simulink model "Three_Phase_Four_Leg_Inverter"  (R2023b)
settings: Solver=FixedStepAuto  StartTime=0.0  StopTime=0.5  RelTol=1e-3
libraries: spsSeriesRLCBranchLib x11, spsVoltageMeasurementLib x7, spsUniversalBridgeLib x4, spsDCVoltageSourceLib x3, spsCurrentMeasurementLib x3, spsRMSLib x2, simulink x1, spsMeanLib x1, spsTHDLib x1, spspowerguiLib x1
settings Model: SimulationMode=accelerator  Creator=abc6820292  LastModifiedBy=Qu
settings SolverCC: ZeroCrossAlgorithm=Adaptive
settings DataIOCC: ReturnWorkspaceOutputs=off  Refine=10
settings DebuggingCC: IgnoredZcDiagnostic=none  UnconnectedInputMsg=warning  UnconnectedOutputMsg=warning  UnconnectedLineMsg=warning
settings ModelReferenceCC: EnableRefExpFcnMdlSchedulingChecks=on
settings RTWCC: DLArmComputeVersion=19.05

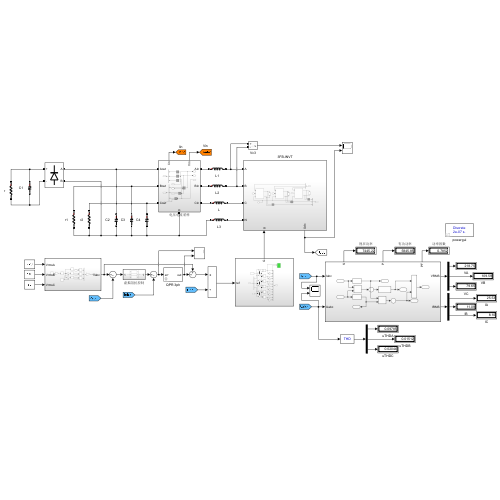
[thumbnail: Simulink's stored preview of the top-level diagram]
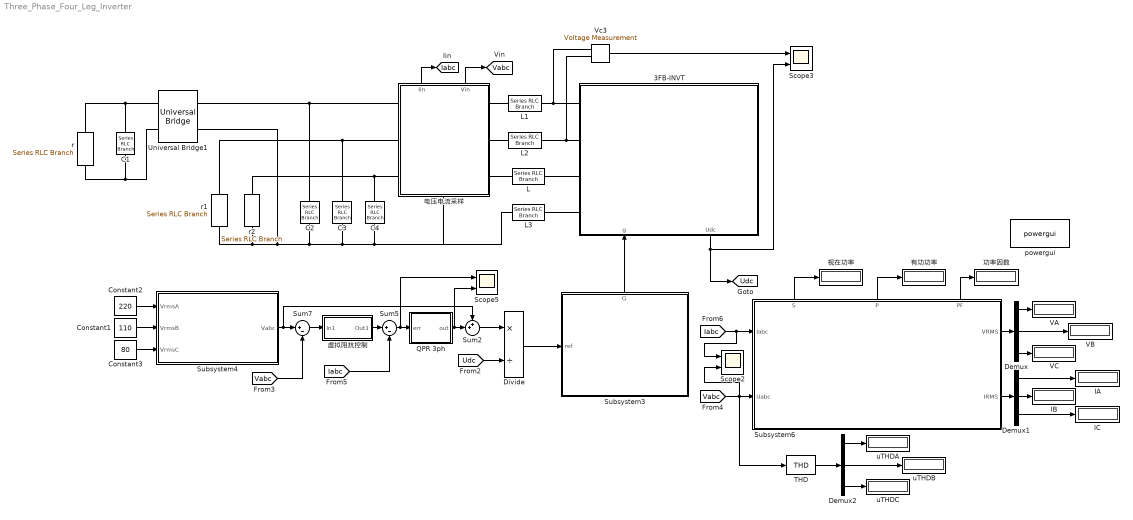
== system Three_Phase_Four_Leg_Inverter ==
  3FB-INVT : Subsystem
      settings: PortSchema="{\"entries\":[{\"content\":{\"sides\":[{\"content\":{\"connectorIds\":[\"LConn1\",\"LConn2\",\"LConn3\",\"LConn4\"]},\"type\":\"ConnectorPlacement.EquallySpacedRectSide\",\"uuid\":\"b14efc91-6835-4ed7-8c1d-e2670cf7c179\"},{\"content\":{\"side\":\"RIGHT\"},\"type\":\"ConnectorPlacement.EquallySpacedRectSide\",\"uuid\":\"133f26b8-b252-4d3c-80df-0b09760e0c14\"},{\"content\":{\"side\":\"TOP\"},\"type\":\"ConnectorPlacement.EquallySpacedRectSide\",\"uuid\":\"c058e102-7791-48c2-b9e4-e80cedcfd34e\"},{\"content\":{\"connectorIds\":[\"In1\",\"Out1\"],\"side\":\"BOTTOM\"},\"type\":\"ConnectorPlacement.EquallySpacedRectSide\",\"uuid\":\"7bcd8845-3331-4b31-8039-611891643c20\"}]},\"type\":\"ConnectorPlacement.EquallySpacedConnector\",\"uuid\":\"173e4324-58a1-473c-9df3-d0606e4a673f\"}],\"packageUris\":[\"http://schema.mathworks.com/mf0/Connector/R2020b\"],\"version\":\"1.0\"}"
  C1 : spsSeriesRLCBranchLib/Series RLC Branch  LConnTagsString=__new0  RConnTagsString=__new0  BranchType=C  Resistance=0  Inductance=0  SetiL0=off  InitialCurrent=0  Capacitance=5e-3  Setx0=on  InitialVoltage=310  Measurements=None
  C2 : spsSeriesRLCBranchLib/Series RLC Branch  LConnTagsString=__new0  RConnTagsString=__new0  BranchType=C  Resistance=0  Inductance=0  SetiL0=off  InitialCurrent=0  Capacitance=5e-6  Setx0=off  InitialVoltage=310  Measurements=None
  C3 : spsSeriesRLCBranchLib/Series RLC Branch  LConnTagsString=__new0  RConnTagsString=__new0  BranchType=C  Resistance=0  Inductance=0  SetiL0=off  InitialCurrent=0  Capacitance=5e-6  Setx0=off  InitialVoltage=310  Measurements=None
  C4 : spsSeriesRLCBranchLib/Series RLC Branch  LConnTagsString=__new0  RConnTagsString=__new0  BranchType=C  Resistance=0  Inductance=0  SetiL0=off  InitialCurrent=0  Capacitance=5e-6  Setx0=off  InitialVoltage=310  Measurements=None
  Constant1 : Constant  Value=110
  Constant2 : Constant  Value=220
  Constant3 : Constant  Value=80
  Demux : Demux  Outputs=3
  Demux1 : Demux  Outputs=3
  Demux2 : Demux  Outputs=3
  Divide : Product  Inputs=*/
  IA : Display
      settings: Format=bank
  IB : Display
      settings: Format=bank
  IC : Display
      settings: Format=bank
  L : spsSeriesRLCBranchLib/Series RLC Branch  LConnTagsString=__new0  RConnTagsString=__new0  BranchType=L  Resistance=1  Inductance=2e-4  SetiL0=off  InitialCurrent=0  Capacitance=inf  Setx0=off  InitialVoltage=0  Measurements=None
  L1 : spsSeriesRLCBranchLib/Series RLC Branch  LConnTagsString=__new0  RConnTagsString=__new0  BranchType=L  Resistance=1  Inductance=2e-4  SetiL0=off  InitialCurrent=0  Capacitance=inf  Setx0=off  InitialVoltage=0  Measurements=None
  L2 : spsSeriesRLCBranchLib/Series RLC Branch  LConnTagsString=__new0  RConnTagsString=__new0  BranchType=L  Resistance=1  Inductance=2e-4  SetiL0=off  InitialCurrent=0  Capacitance=inf  Setx0=off  InitialVoltage=0  Measurements=None
  L3 : spsSeriesRLCBranchLib/Series RLC Branch  LConnTagsString=__new0  RConnTagsString=__new0  BranchType=L  Resistance=0.01  Inductance=2e-4  SetiL0=off  InitialCurrent=0  Capacitance=inf  Setx0=off  InitialVoltage=0  Measurements=None
  QPR 3ph : Subsystem  mask{Kp=8, Kr=100, Wc=5, Ts=1/30000, Upper=600, Lower=-600}
      mask DialogControl ParameterGroupVar Prompt: 参数
  Scope2 : Scope  NumInputPorts=2
  Scope3 : Scope  NumInputPorts=2
  Scope5 : Scope  NumInputPorts=2
  Subsystem3 : Subsystem
      settings: PortSchema="{\"entries\":[{\"content\":{\"sides\":[{\"content\":{\"connectorIds\":[\"In1\"]},\"type\":\"ConnectorPlacement.EquallySpacedRectSide\",\"uuid\":\"86d8a801-af54-4615-919a-9a70996995f5\"},{\"content\":{\"side\":\"RIGHT\"},\"type\":\"ConnectorPlacement.EquallySpacedRectSide\",\"uuid\":\"9c099dd5-197a-4a29-8cd5-6822de601230\"},{\"content\":{\"connectorIds\":[\"Out1\"],\"side\":\"TOP\"},\"type\":\"ConnectorPlacement.EquallySpacedRectSide\",\"uuid\":\"5852d946-2383-4602-be71-32d16fa24bc3\"}]},\"type\":\"ConnectorPlacement.EquallySpacedConnector\",\"uuid\":\"a21c857f-e780-49b2-9a65-1676cf4540b1\"}],\"packageUris\":[\"http://schema.mathworks.com/mf0/Connector/R2020b\"],\"version\":\"1.0\"}"
  Subsystem4 : Subsystem
  Subsystem6 : Subsystem
      settings: PortSchema="{\"entries\":[{\"content\":{\"sides\":[{\"content\":{\"connectorIds\":[\"In1\",\"In2\"]},\"type\":\"ConnectorPlacement.EquallySpacedRectSide\",\"uuid\":\"8f3b7bf1-7c44-4492-a357-aa6e3e6d66a4\"},{\"content\":{\"connectorIds\":[\"Out1\",\"Out2\"],\"side\":\"RIGHT\"},\"type\":\"ConnectorPlacement.EquallySpacedRectSide\",\"uuid\":\"7ae784cf-6bcf-4684-9c07-1770fc60c8a0\"},{\"content\":{\"connectorIds\":[\"Out3\",\"Out4\",\"Out5\"],\"side\":\"TOP\"},\"type\":\"ConnectorPlacement.EquallySpacedRectSide\",\"uuid\":\"0e016931-6232-4ad6-afe9-572a0571336f\"},{\"content\":{\"side\":\"BOTTOM\"},\"type\":\"ConnectorPlacement.EquallySpacedRectSide\",\"uuid\":\"ef67c6ee-ba81-4705-af34-81581e7e9907\"}]},\"type\":\"ConnectorPlacement.EquallySpacedConnector\",\"uuid\":\"922af512-c0ff-443f-816c-194775a78dc8\"}],\"packageUris\":[\"http://schema.mathworks.com/mf0/Connector/R2020b\"],\"version\":\"1.0\"}"
  Sum2 : Sum  Inputs=++|
  Sum5 : Sum  Inputs=|+-
  Sum7 : Sum  Inputs=|+-
  THD : spsTHDLib/THD  Freq=50  Ts=0
  Universal Bridge1 : spsUniversalBridgeLib/Universal Bridge  Arms=2  SnubberResistance=1e6  SnubberCapacitance=inf  Device=Diodes  Ron=1e-3  Lon=0  ForwardVoltages="[  1  1  ]"  ForwardVoltage=1  GTOparameters=[ 10e-6 , 20e-6 ]  IGBTparameters=[ 1e-6 , 2e-6 ]  Measurements=None  Measurements_2=None  converterType=Rectifier
  VA : Display
      settings: Format=bank
  VB : Display
      settings: Format=bank
  VC : Display
      settings: Format=bank
  Vc3 : spsVoltageMeasurementLib/Voltage Measurement  PhasorSimulation=off  OutputType=Complex  PSBequivalent=0
  powergui : spspowerguiLib/powergui  Priority=1  SimulationMode=Discrete  SampleTime=2e-7  frequency=60  Iterations=50  frequencyindice=0  Pbase=100e6  ErrMax=1e-4  UnitsV=kV  UnitsW=MW  buscounter=0  FunctionMessages=off  echomessages=off  EnableUseOfTLC=off  CurrentSourceSwitches=off  DisableSnubberDevices=off  DisableRonSwitches=off  DisableVfSwitches=off  DisplayEquations=off  AutomaticDiscreteSolvers=off  SolverType=Tustin/Backward Euler (TBE)  Interpol=off  ExternalGateDelay=off  methode=off  Ts=100  x0status=blocks  SPID=on  SwTol=0  HookPort=off  NonlinearTolerance=1e-4  nMaxIteration=100  ContinueOnMaxIteration=off  RestoreLinks=warning  ResistiveCurrentMeasurement=off  Frange=[0:2:500]  Ylog=off  Xlog=on  ShowGrid=off  save=off  variable=ZData  structure=0  ZoomFFT=off  StartTime=0.0  cycles=1  DisplayStyle=1  fundamental=60  FreqAxis=off  MaxFrequency=1000  frequencyindicesteady=1  RmsSteady=1  display=off
  r : spsSeriesRLCBranchLib/Series RLC Branch  LConnTagsString=__new0  RConnTagsString=__new0  BranchType=R  Resistance=30  Inductance=12e-4  SetiL0=off  InitialCurrent=0  Capacitance=inf  Setx0=off  InitialVoltage=0  Measurements=None
  r1 : spsSeriesRLCBranchLib/Series RLC Branch  LConnTagsString=__new0  RConnTagsString=__new0  BranchType=R  Resistance=10  Inductance=12e-4  SetiL0=off  InitialCurrent=0  Capacitance=inf  Setx0=off  InitialVoltage=0  Measurements=None
  r2 : spsSeriesRLCBranchLib/Series RLC Branch  LConnTagsString=__new0  RConnTagsString=__new0  BranchType=R  Resistance=10  Inductance=12e-4  SetiL0=off  InitialCurrent=0  Capacitance=inf  Setx0=off  InitialVoltage=0  Measurements=None
  uTHDA : Display
  uTHDB : Display
  uTHDC : Display
  功率因数 : Display
  有功功率 : Display
      settings: Format=bank
  电压电流采样 : Subsystem
      settings: PortSchema="{\"entries\":[{\"content\":{\"sides\":[{\"content\":{\"connectorIds\":[\"LConn1\",\"LConn2\",\"LConn3\"]},\"type\":\"ConnectorPlacement.EquallySpacedRectSide\",\"uuid\":\"d60dd16a-7a74-435a-96f5-79c0993f3801\"},{\"content\":{\"connectorIds\":[\"RConn1\",\"RConn2\",\"RConn3\"],\"side\":\"RIGHT\"},\"type\":\"ConnectorPlacement.EquallySpacedRectSide\",\"uuid\":\"38a0d536-50a5-43bd-9d58-6b0db9c378a0\"},{\"content\":{\"connectorIds\":[\"Out1\",\"Out2\"],\"side\":\"TOP\"},\"type\":\"ConnectorPlacement.EquallySpacedRectSide\",\"uuid\":\"65be575f-dbb8-4f94-beb1-b426df65c1d5\"},{\"content\":{\"connectorIds\":[\"RConn4\"],\"side\":\"BOTTOM\"},\"type\":\"ConnectorPlacement.EquallySpacedRectSide\",\"uuid\":\"a28dffe8-15db-4523-b673-2414d0fbe1e1\"}]},\"type\":\"ConnectorPlacement.EquallySpacedConnector\",\"uuid\":\"1fc3ca7a-50b1-4fd5-a5d3-d39cc1e6f07d\"}],\"packageUris\":[\"http://schema.mathworks.com/mf0/Connector/R2020b\"],\"version\":\"1.0\"}"
  虚拟阻抗控制 : Subsystem
  视在功率 : Display
      settings: Format=bank
  tag scope: Iabc=global, Udc=global, Vabc=global
  wires:
  Vc3/1 -> Scope3/1
  3FB-INVT/1(Udc) -> [Udc], Scope3/2
  Subsystem3/1(G) -> 3FB-INVT/1(g)
  Demux/3 -> VC/1
  [Udc] -> Divide/2
  Sum2/1 -> Divide/1
  Demux2/1 -> uTHDA/1
  Subsystem6/3(S) -> 视在功率/1
  Demux/1 -> VA/1
  [Vabc] -> THD/1, Scope2/2, Subsystem6/2(Uabc)
  Subsystem6/1(VRMS) -> Demux/1
  QPR 3ph/1(out) -> Scope5/2, Sum2/2
  Demux2/3 -> uTHDC/1
  Demux1/1 -> IA/1
  Divide/1 -> Subsystem3/1(ref)
  Demux/2 -> VB/1
  Demux1/3 -> IC/1
  虚拟阻抗控制/1(Out1) -> Sum5/1
  THD/1 -> Demux2/1
  Subsystem6/5(PF) -> 功率因数/1
  Subsystem6/4(P) -> 有功功率/1
  Demux2/2 -> uTHDB/1
  Demux1/2 -> IB/1
  Subsystem4/1(Vabc) -> Sum2/1, Sum7/1
  Subsystem6/2(IRMS) -> Demux1/1
  [Iabc] -> Scope2/1, Subsystem6/1(Iabc)
  Sum5/1 -> Scope5/1, QPR 3ph/1(err)
  Constant2/1 -> Subsystem4/1(VrmsA)
  Sum7/1 -> 虚拟阻抗控制/1(In1)
  [Vabc] -> Sum7/2
  [Iabc] -> Sum5/2
  电压电流采样/1(Vin) -> [Vabc]
  电压电流采样/2(Iin) -> [Iabc]
  Constant1/1 -> Subsystem4/2(VrmsB)
  Constant3/1 -> Subsystem4/3(VrmsC)
  connections:
  C3/LConn1 -- 电压电流采样/RConn2 -- r1/LConn1
  r2/RConn1 -- r1/RConn1 -- Universal Bridge1/LConn2 -- C4/RConn1 -- 电压电流采样/RConn4 -- L3/LConn1 -- C3/RConn1 -- C2/RConn1
  L1/RConn1 -- Vc3/LConn1 -- 3FB-INVT/LConn1
  C2/LConn1 -- 电压电流采样/RConn1 -- Universal Bridge1/LConn1
  L2/RConn1 -- Vc3/LConn2 -- 3FB-INVT/LConn2
  C4/LConn1 -- 电压电流采样/RConn3 -- r2/LConn1
  电压电流采样/LConn2 -- L2/LConn1
  L/RConn1 -- 3FB-INVT/LConn3
  电压电流采样/LConn1 -- L1/LConn1
  电压电流采样/LConn3 -- L/LConn1
  L3/RConn1 -- 3FB-INVT/LConn4
  Universal Bridge1/RConn1 -- C1/LConn1 -- r/LConn1
  Universal Bridge1/RConn2 -- C1/RConn1 -- r/RConn1

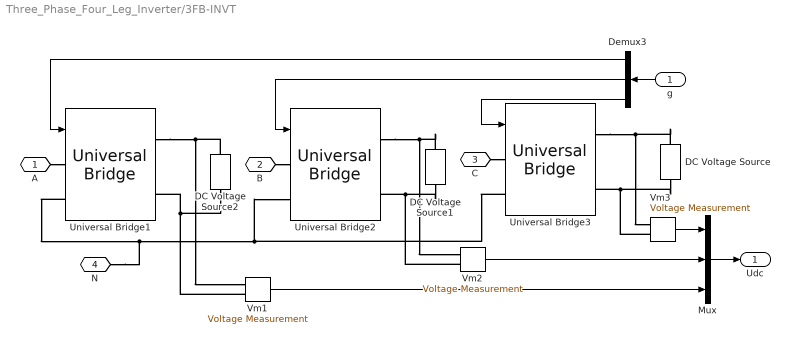
== system Three_Phase_Four_Leg_Inverter/3FB-INVT ==
  g : Inport
  DC Voltage Source : spsDCVoltageSourceLib/DC Voltage Source  Amplitude=375  Measurements=None
  DC Voltage Source1 : spsDCVoltageSourceLib/DC Voltage Source  Amplitude=375  Measurements=None
  DC Voltage Source2 : spsDCVoltageSourceLib/DC Voltage Source  Amplitude=375  Measurements=None
  Demux3 : Demux  Outputs=3
  Mux : Mux  Inputs=3
  Universal Bridge1 : spsUniversalBridgeLib/Universal Bridge  Arms=2  SnubberResistance=1e6  SnubberCapacitance=inf  Device=IGBT / Diodes  Ron=1e-3  Lon=0  ForwardVoltages="[  1  1  ]"  ForwardVoltage=0  GTOparameters=[ 10e-6 , 20e-6 ]  IGBTparameters=[ 1e-6 , 2e-6 ]  Measurements=None  Measurements_2=None  converterType=Rectifier
  Universal Bridge2 : spsUniversalBridgeLib/Universal Bridge  Arms=2  SnubberResistance=1e6  SnubberCapacitance=inf  Device=IGBT / Diodes  Ron=1e-3  Lon=0  ForwardVoltages="[  1  1  ]"  ForwardVoltage=0  GTOparameters=[ 10e-6 , 20e-6 ]  IGBTparameters=[ 1e-6 , 2e-6 ]  Measurements=None  Measurements_2=None  converterType=Rectifier
  Universal Bridge3 : spsUniversalBridgeLib/Universal Bridge  Arms=2  SnubberResistance=1e6  SnubberCapacitance=inf  Device=IGBT / Diodes  Ron=1e-3  Lon=0  ForwardVoltages="[  1  1  ]"  ForwardVoltage=0  GTOparameters=[ 10e-6 , 20e-6 ]  IGBTparameters=[ 1e-6 , 2e-6 ]  Measurements=None  Measurements_2=None  converterType=Rectifier
  Vm1 : spsVoltageMeasurementLib/Voltage Measurement  PhasorSimulation=off  OutputType=Complex  PSBequivalent=0
  Vm2 : spsVoltageMeasurementLib/Voltage Measurement  PhasorSimulation=off  OutputType=Complex  PSBequivalent=0
  Vm3 : spsVoltageMeasurementLib/Voltage Measurement  PhasorSimulation=off  OutputType=Complex  PSBequivalent=0
  A : PMIOPort  Side=Left
  B : PMIOPort  Port=2  Side=Left
  C : PMIOPort  Port=3  Side=Left
  N : PMIOPort  Port=4  Side=Left
  Udc : Outport
  wires:
  g/1 -> Demux3/1
  Vm3/1 -> Mux/1
  Vm2/1 -> Mux/2
  Vm1/1 -> Mux/3
  Demux3/3 -> Universal Bridge3/1
  Demux3/2 -> Universal Bridge2/1
  Demux3/1 -> Universal Bridge1/1
  Mux/1 -> Udc/1
  connections:
  Universal Bridge1/RConn1 -- DC Voltage Source2/RConn1 -- Vm1/LConn1
  Vm1/LConn2 -- Universal Bridge1/RConn2 -- DC Voltage Source2/LConn1
  A/RConn1 -- Universal Bridge1/LConn1
  Universal Bridge2/RConn1 -- DC Voltage Source1/RConn1 -- Vm2/LConn1
  Vm2/LConn2 -- DC Voltage Source1/LConn1 -- Universal Bridge2/RConn2
  Universal Bridge3/RConn1 -- DC Voltage Source/RConn1 -- Vm3/LConn1
  Vm3/LConn2 -- Universal Bridge3/RConn2 -- DC Voltage Source/LConn1
  B/RConn1 -- Universal Bridge2/LConn1
  C/RConn1 -- Universal Bridge3/LConn1
  Universal Bridge1/LConn2 -- N/RConn1 -- Universal Bridge3/LConn2 -- Universal Bridge2/LConn2

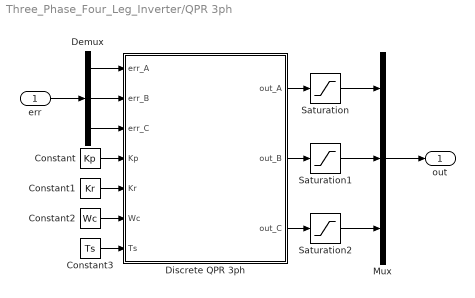
== system Three_Phase_Four_Leg_Inverter/QPR 3ph ==
  err : Inport
  Constant : Constant  Value=Kp
  Constant1 : Constant  Value=Kr
  Constant2 : Constant  Value=Wc
  Constant3 : Constant  Value=Ts
  Demux : Demux  Outputs=3
  Discrete QPR 3ph : MATLAB Function  TreatAsAtomicUnit=on
  Mux : Mux  Inputs=3
  Saturation : Saturate  UpperLimit=Upper  LowerLimit=Lower
  Saturation1 : Saturate  UpperLimit=Upper  LowerLimit=Lower
  Saturation2 : Saturate  UpperLimit=Upper  LowerLimit=Lower
  out : Outport
  wires:
  Discrete QPR 3ph/1(out_A) -> Saturation/1
  Constant1/1 -> Discrete QPR 3ph/5(Kr)
  Constant3/1 -> Discrete QPR 3ph/7(Ts)
  Constant/1 -> Discrete QPR 3ph/4(Kp)
  Constant2/1 -> Discrete QPR 3ph/6(Wc)
  Discrete QPR 3ph/2(out_B) -> Saturation1/1
  Discrete QPR 3ph/3(out_C) -> Saturation2/1
  Demux/2 -> Discrete QPR 3ph/2(err_B)
  Demux/3 -> Discrete QPR 3ph/3(err_C)
  Demux/1 -> Discrete QPR 3ph/1(err_A)
  err/1 -> Demux/1
  Saturation2/1 -> Mux/3
  Saturation1/1 -> Mux/2
  Saturation/1 -> Mux/1
  Mux/1 -> out/1

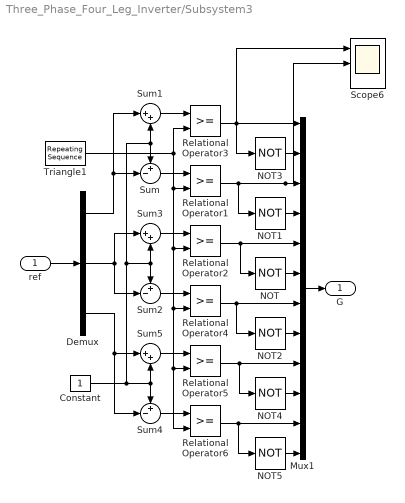
== system Three_Phase_Four_Leg_Inverter/Subsystem3 ==
  ref : Inport
  Constant : Constant
  Demux : Demux  Outputs=3
  Mux1 : Mux  Inputs=12
  NOT{,1..5} (6 alike) : Logic  Operator=NOT  IconShape=distinctive  AllPortsSameDT=off  OutDataTypeStr=boolean
  Relational Operator{1..6} (6 alike) : RelationalOperator  OutDataTypeStr=boolean  InputSameDT=off
  Scope6 : Scope  NumInputPorts=3
  Sum : Sum  Inputs=+-|
  Sum1 : Sum  Inputs=|++
  Sum2 : Sum  Inputs=+-|
  Sum3 : Sum  Inputs=|++
  Sum4 : Sum  Inputs=+-|
  Sum5 : Sum  Inputs=|++
  Triangle1 : simulink/Sources/Repeating Sequence  rep_seq_t=[0 1/30000/2 1/30000]  rep_seq_y=[0 2 0]
  G : Outport
  wires:
  Relational Operator2/1 -> Mux1/5, NOT/1
  Relational Operator3/1 -> NOT3/1, Scope6/1, Mux1/1
  Mux1/1 -> G/1
  Relational Operator5/1 -> Mux1/9, NOT4/1
  Relational Operator6/1 -> Mux1/11, NOT5/1
  NOT3/1 -> Mux1/2
  NOT/1 -> Mux1/6
  NOT4/1 -> Mux1/10
  Triangle1/1 -> Relational Operator6/2, Relational Operator5/2, Relational Operator4/2, Relational Operator2/2, Relational Operator1/2, Relational Operator3/2
  Sum/1 -> Relational Operator1/1
  Demux/1 -> Sum1/1, Sum/2
  Sum1/1 -> Relational Operator3/1
  Constant/1 -> Sum/1, Sum1/2, Sum3/2, Sum2/1, Sum5/2, Sum4/1
  Demux/2 -> Sum2/2, Sum3/1
  Sum3/1 -> Relational Operator2/1
  Sum2/1 -> Relational Operator4/1
  Sum5/1 -> Relational Operator5/1
  Sum4/1 -> Relational Operator6/1
  Demux/3 -> Sum4/2, Sum5/1
  NOT5/1 -> Mux1/12
  NOT2/1 -> Mux1/8
  Relational Operator4/1 -> NOT2/1, Mux1/7
  NOT1/1 -> Mux1/4
  Relational Operator1/1 -> Scope6/2, Mux1/3, NOT1/1
  ref/1 -> Demux/1

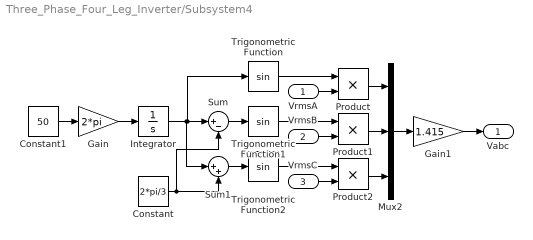
== system Three_Phase_Four_Leg_Inverter/Subsystem4 ==
  VrmsA : Inport
  VrmsB : Inport  Port=2
  VrmsC : Inport  Port=3
  Constant : Constant  Value=2*pi/3
  Constant1 : Constant  Value=50
  Gain : Gain  Gain=2*pi
  Gain1 : Gain  Gain=1.415
  Integrator : Integrator  WrapState=on  WrappedStateUpperValue=2*pi  WrappedStateLowerValue=0
  Mux2 : Mux  Inputs=3
  Product : Product
  Product1 : Product
  Product2 : Product
  Sum : Sum  Inputs=|+-
  Sum1 : Sum  Inputs=|++
  Trigonometric Function : Trigonometry
  Trigonometric Function1 : Trigonometry
  Trigonometric Function2 : Trigonometry
  Vabc : Outport
  wires:
  Gain/1 -> Integrator/1
  Integrator/1 -> Sum1/1, Trigonometric Function/1, Sum/1
  Constant/1 -> Sum1/2, Sum/2
  Sum/1 -> Trigonometric Function1/1
  Sum1/1 -> Trigonometric Function2/1
  Constant1/1 -> Gain/1
  Trigonometric Function/1 -> Product/1
  Product/1 -> Mux2/1
  Trigonometric Function1/1 -> Product1/1
  Product1/1 -> Mux2/2
  Trigonometric Function2/1 -> Product2/1
  Product2/1 -> Mux2/3
  Mux2/1 -> Gain1/1
  Gain1/1 -> Vabc/1
  VrmsA/1 -> Product/2
  VrmsC/1 -> Product2/2
  VrmsB/1 -> Product1/2

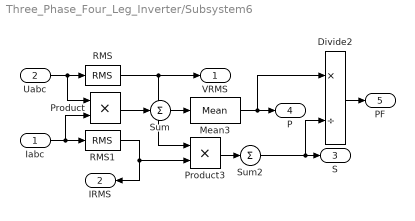
== system Three_Phase_Four_Leg_Inverter/Subsystem6 ==
  Iabc : Inport
  Uabc : Inport  Port=2
  Divide2 : Product  Inputs=*/
  Mean3 : spsMeanLib/Mean  Freq=50  Vinit=0  Ts=0
  Product : Product
  Product3 : Product
  RMS : spsRMSLib/RMS  TrueRMS=on  Freq=50  RMSInit=0  Ts=0
  RMS1 : spsRMSLib/RMS  TrueRMS=on  Freq=50  RMSInit=0  Ts=0
  Sum : Sum  Inputs=+
  Sum2 : Sum  Inputs=+
  VRMS : Outport
  IRMS : Outport  Port=2
  S : Outport  Port=3
  P : Outport  Port=4
  PF : Outport  Port=5
  wires:
  Iabc/1 -> Product/2, RMS1/1
  RMS/1 -> VRMS/1, Product3/1
  RMS1/1 -> Product3/2, IRMS/1
  Divide2/1 -> PF/1
  Mean3/1 -> Divide2/1, P/1
  Sum/1 -> Mean3/1
  Uabc/1 -> RMS/1, Product/1
  Product/1 -> Sum/1
  Product3/1 -> Sum2/1
  Sum2/1 -> Divide2/2, S/1

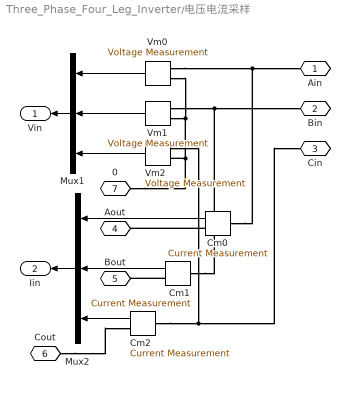
== system Three_Phase_Four_Leg_Inverter/电压电流采样 ==
  Cm0 : spsCurrentMeasurementLib/Current Measurement  PhasorSimulation=off  OutputType=Complex  PSBequivalent=0
  Cm1 : spsCurrentMeasurementLib/Current Measurement  PhasorSimulation=off  OutputType=Complex  PSBequivalent=0
  Cm2 : spsCurrentMeasurementLib/Current Measurement  PhasorSimulation=off  OutputType=Complex  PSBequivalent=0
  Mux1 : Mux  Inputs=3
  Mux2 : Mux  Inputs=3
  Vm0 : spsVoltageMeasurementLib/Voltage Measurement  PhasorSimulation=off  OutputType=Complex  PSBequivalent=0
  Vm1 : spsVoltageMeasurementLib/Voltage Measurement  PhasorSimulation=off  OutputType=Complex  PSBequivalent=0
  Vm2 : spsVoltageMeasurementLib/Voltage Measurement  PhasorSimulation=off  OutputType=Complex  PSBequivalent=0
  Ain : PMIOPort  Side=Left
  Bin : PMIOPort  Port=2  Side=Left
  Cin : PMIOPort  Port=3  Side=Left
  Aout : PMIOPort  Port=4  Side=Right
  Bout : PMIOPort  Port=5  Side=Right
  Cout : PMIOPort  Port=6  Side=Right
  0 : PMIOPort  Port=7  Side=Right
  Vin : Outport
  Iin : Outport  Port=2
  wires:
  Cm2/1 -> Mux2/3
  Vm1/1 -> Mux1/2
  Cm1/1 -> Mux2/2
  Vm2/1 -> Mux1/3
  Vm0/1 -> Mux1/1
  Mux1/1 -> Vin/1
  Cm0/1 -> Mux2/1
  Mux2/1 -> Iin/1
  connections:
  Vm1/LConn1 -- Cm1/LConn1 -- Bin/RConn1
  Cm0/RConn1 -- Aout/RConn1
  Vm0/LConn1 -- Cm0/LConn1 -- Ain/RConn1
  Cm2/LConn1 -- Vm2/LConn1 -- Cin/RConn1
  Cm1/RConn1 -- Bout/RConn1
  Cout/RConn1 -- Cm2/RConn1
  0/RConn1 -- Vm0/LConn2 -- Vm1/LConn2 -- Vm2/LConn2

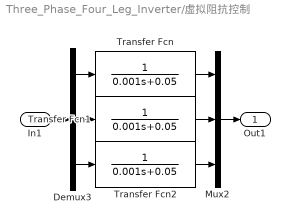
== system Three_Phase_Four_Leg_Inverter/虚拟阻抗控制 ==
  In1 : Inport
  Demux3 : Demux  Outputs=3
  Mux2 : Mux  Inputs=3
  Transfer Fcn : TransferFcn  Denominator=[0.001 0.05]
  Transfer Fcn1 : TransferFcn  Denominator=[0.001 0.05]
  Transfer Fcn2 : TransferFcn  Denominator=[0.001 0.05]
  Out1 : Outport
  wires:
  Demux3/2 -> Transfer Fcn1/1
  Transfer Fcn/1 -> Mux2/1
  Mux2/1 -> Out1/1
  Transfer Fcn1/1 -> Mux2/2
  Transfer Fcn2/1 -> Mux2/3
  Demux3/3 -> Transfer Fcn2/1
  Demux3/1 -> Transfer Fcn/1
  In1/1 -> Demux3/1

== matlab function Three_Phase_Four_Leg_Inverter/QPR 3ph/Discrete QPR 3ph ==
  settings: updateMethod=DISCRETE  sampleTime=Ts
  data: err_A input; err_B input; err_C input; out_A output; Kp input; Kr input; Wc input; Ts input; out_B output; out_C output
function [out_A, out_B, out_C] = fcn(err_A, err_B, err_C, Kp, Kr, Wc, Ts)

W0 = 50*2*pi;

%%定义三相静态变量
persistent err_A1;
persistent err_A2;
persistent out_A1;
persistent out_A2;

persistent err_B1;
persistent err_B2;
persistent out_B1;
persistent out_B2;

persistent err_C1;
persistent err_C2;
persistent out_C1;
persistent out_C2;

%%对三相静态变量初始化
if isempty(err_A1)
    err_A1 = 0;
end
if isempty(err_A2)
    err_A2 = 0;
end
if isempty(out_A1)
    out_A1 = 0;
end
if isempty(out_A2)
    out_A2 = 0;
end

if isempty(err_B1)
    err_B1 = 0;
end
if isempty(err_B2)
    err_B2 = 0;
end
if isempty(out_B1)
    out_B1 = 0;
end
if isempty(out_B2)
    out_B2 = 0;
end

if isempty(err_C1)
    err_C1 = 0;
end
if isempty(err_C2)
    err_C2 = 0;
end
if isempty(out_C1)
    out_C1 = 0;
end
if isempty(out_C2)
    out_C2 = 0;
end

%%Discrete
t1 = Wc * Ts;
t2 = W0^2 * Ts^2;
t3 = t2 + 4*t1 + 4;

b0 = (Kp*t2 + 4*(Kp+Kr)*t1 + 4*Kp) / t3;
b1 = (2*Kp*t2 - 8*Kp) / t3;
b2 = (Kp*t2 + 4*Kp - 4*(Kp+Kr)*t1) / t3;
a1 = (2*t2 - 8) / t3;
a2 = (t2 - 4*t1 + 4) / t3;

%%计算三相输出量
out_A = b0*err_A + b1*err_A1 + b2*err_A2 - a1*out_A1 - a2*out_A2;
out_A2 = out_A1;
out_A1 = out_A;
err_A2 = err_A1;
err_A1 = err_A;

out_B = b0*err_B + b1*err_B1 + b2*err_B2 - a1*out_B1 - a2*out_B2;
out_B2 = out_B1;
out_B1 = out_B;
err_B2 = err_B1;
err_B1 = err_B;

out_C = b0*err_C + b1*err_C1 + b2*err_C2 - a1*out_C1 - a2*out_C2;
out_C2 = out_C1;
out_C1 = out_C;
err_C2 = err_C1;
err_C1 = err_C;
